simulink model "test_motion_controller"  (R2025a)
settings: Solver=FixedStepAuto  StartTime=0.0  StopTime=5  RelTol=1e-3
model workspace (MAT data in the model file):
  InitConfParams = Simulink.Parameter
  InitConfParams.Value.thresholds.jntVelMax = 40000
  InitConfParams.Value.thresholds.motorNominalCurrents = 0.34999999404
  InitConfParams.Value.thresholds.motorPeakCurrents = 0.699999988079
  InitConfParams.Value.thresholds.motorOverloadCurrents = 1
  InitConfParams.Value.thresholds.motorPwmLimit = 32000
  InitConfParams.Value.thresholds.motorCriticalTemperature = 0
  InitConfParams.Value.pids.currentPID.type : enumeration (value not decoded)
  InitConfParams.Value.pids.currentPID.OutMax = 0
  InitConfParams.Value.pids.currentPID.OutMin = 0
  InitConfParams.Value.pids.currentPID.P = 2
  InitConfParams.Value.pids.currentPID.I = 500
  InitConfParams.Value.pids.currentPID.D = 0
  InitConfParams.Value.pids.currentPID.N = 10
  InitConfParams.Value.pids.currentPID.I0 = 0
  InitConfParams.Value.pids.currentPID.D0 = 0
  InitConfParams.Value.pids.currentPID.shift_factor = 0
  InitConfParams.Value.pids.velocityPID.type : enumeration (value not decoded)
  InitConfParams.Value.pids.velocityPID.OutMax = 0
  InitConfParams.Value.pids.velocityPID.OutMin = 0
  InitConfParams.Value.pids.velocityPID.P = -20
  InitConfParams.Value.pids.velocityPID.I = -20
  InitConfParams.Value.pids.velocityPID.D = 0
  InitConfParams.Value.pids.velocityPID.N = 100
  InitConfParams.Value.pids.velocityPID.I0 = 0
  InitConfParams.Value.pids.velocityPID.D0 = 0
  InitConfParams.Value.pids.velocityPID.shift_factor = 10
  InitConfParams.Value.pids.positionPID.type : enumeration (value not decoded)
  InitConfParams.Value.pids.positionPID.OutMax = 0
  InitConfParams.Value.pids.positionPID.OutMin = 0
  InitConfParams.Value.pids.positionPID.P = 0
  InitConfParams.Value.pids.positionPID.I = 0
  InitConfParams.Value.pids.positionPID.D = 0
  InitConfParams.Value.pids.positionPID.N = 0
  InitConfParams.Value.pids.positionPID.I0 = 0
  InitConfParams.Value.pids.positionPID.D0 = 0
  InitConfParams.Value.pids.positionPID.shift_factor = 0
  InitConfParams.Value.motor.externals.enable_verbosity = 0
  InitConfParams.Value.motor.externals.has_hall_sens = 1
  InitConfParams.Value.motor.externals.has_quadrature_encoder = 0
  InitConfParams.Value.motor.externals.has_speed_quadrature_encoder = 0
  InitConfParams.Value.motor.externals.has_temperature_sens = 0
  InitConfParams.Value.motor.externals.encoder_tolerance = 0
  InitConfParams.Value.motor.externals.pole_pairs = 7
  InitConfParams.Value.motor.externals.rotor_encoder_resolution = 0
  InitConfParams.Value.motor.externals.rotor_index_offset = 0
  InitConfParams.Value.motor.externals.use_index = 0
  InitConfParams.Value.motor.Kbemf = 0
  InitConfParams.Value.motor.Rphase = 0
  InitConfParams.Value.motor.Imin = 0
  InitConfParams.Value.motor.Imax = 0
  InitConfParams.Value.motor.Vmax = 24
  InitConfParams.Value.motor.resistance = 25.8999996185
  InitConfParams.Value.motor.inductance = 271
  InitConfParams.Value.motor.thermal_resistance = 16
  InitConfParams.Value.motor.thermal_time_constant = 797.5
  InitConfParams.Value.motor.hall_sensors_offset = 30
  InitConfParams.Complexity = 'real'
  InitConfParams.Dimensions = [1 1]
  InitConfParams.DataType = 'Bus: ActuatorConfiguration'
undefined symbols (not defined in the file): ControlModes, EventTypes
settings Model: DataDictionary=embeddedBoard_common.sldd  Creator=mfussi  LastModifiedBy=mfussi
settings SolverCC: ConcurrentTasks=on  AutoInsertRateTranBlk=on
settings DataIOCC: SaveOutput=off  DSMLogging=off  SaveTime=off
settings OptimizationCC: DefaultParameterBehavior=Inlined  EnhancedBackFolding=on  PassReuseOutputArgsAs=Individual arguments  ZeroExternalMemoryAtStartup=off  ZeroInternalMemoryAtStartup=off  SimCompilerOptimization=on  OptimizeBlockOrder=speed  DifferentSizesBufferReuse=on  OptimizationCustomize=off  EfficientTunableParamExpr=on
settings DebuggingCC: ParameterPrecisionLossMsg=none  ParameterTunabilityLossMsg=error
settings ModelReferenceCC: SupportModelReferenceSimTargetCustomCode=on
settings SFSimCC: MATLABDynamicMemAlloc=off  SimTargetLang=C++  SimDLTargetLibrary=mkl-dnn
settings RTWCC: SystemTargetFile=ert.tlc  TemplateMakefile=ert_default_tmf  GPUComputeCapability=3.5  Description=Embedded Coder
settings CodeAppCC: ForceParamTrailComments=on  IgnoreCustomStorageClasses=off  MaxIdLength=95.0  OperatorAnnotations=on  SimulinkDataObjDesc=on  SFDataObjDesc=on  InsertBlockDesc=on
settings ERTTargetCC: ExtModeTransport=0.0  ExtModeStaticAlloc=off  ExtModeMexFile=ext_comm  ExtModeIntrfLevel=Level1  ERTCustomFileTemplate=example_file_process.tlc  TargetLangStandard=C99 (ISO)  GenerateSampleERTMain=on

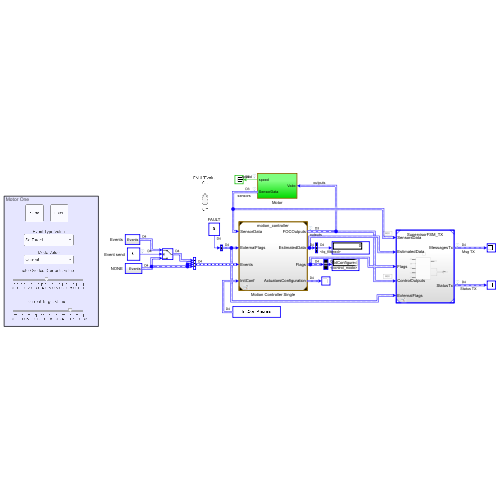
[thumbnail: Simulink's stored preview of the top-level diagram]
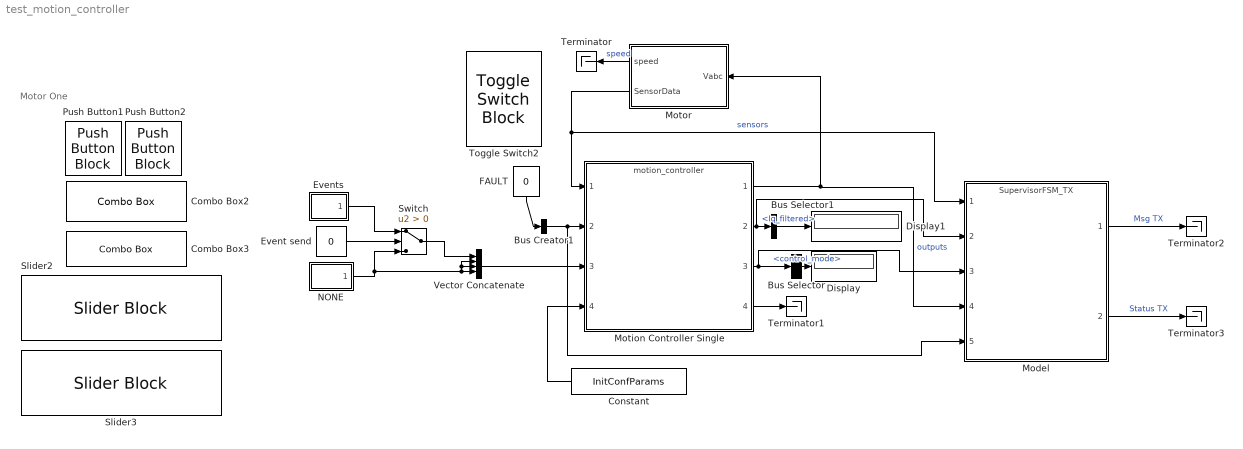
== system test_motion_controller ==
  note: Motor One
  Bus Creator1 : BusCreator  Inputs=1  OutDataTypeStr=Bus: ExternalFlags  NonVirtualBus=on
      settings: InheritFromInputs=off
  Bus Selector : BusSelector  OutputSignals=control_mode
  Bus Selector1 : BusSelector  OutputSignals=Iq_filtered
  Combo Box2 : ComboBox  SelectedLabel=SetTarget  UseEnumeratedDataType=on  EnumeratedDataType=EventTypes
  Combo Box3 : ComboBox  SelectedLabel=Current  UseEnumeratedDataType=on  EnumeratedDataType=ControlModes
  Constant : Constant  Value=InitConfParams  OutDataTypeStr=Bus: ActuatorConfiguration  SampleTime=1e-3
  Display : Display
  Display1 : Display
  Event send : Constant  Value=0  OutDataTypeStr=boolean  SampleTime=1e-3
  Events : Subsystem
  FAULT : Constant  Value=0  OutDataTypeStr=Inherit: Inherit via back propagation  SampleTime=0.001
  Model : ModelReference  ModelNameDialog=SupervisorFSM_TX.slx  SimulationMode=Normal  ModelReferenceVersion=10.14
  Motion Controller Single : ModelReference  ModelNameDialog=motion_controller.slx  ModelReferenceVersion=5.2
  Motor : Subsystem
  NONE : Subsystem
  Push Button1 : PushButtonBlock  ButtonText=Send  IconOnColor=[0.0, 0.39215686274509803, 0.0]  IconOffColor=[0.0, 1.0, 0.0]  OffValue=0.000000
  Push Button2 : PushButtonBlock  ButtonText=Latch  ButtonType=Latch  IconOnColor=[0.0, 0.39215686274509803, 0.0]  IconOffColor=[0.0, 1.0, 0.0]  OffValue=0.000000
  Slider2 : SliderBlock  ScaleMax=1
  Slider3 : SliderBlock  ScaleMax=0.36
  Switch : Switch  Criteria=u2 > Threshold  SaturateOnIntegerOverflow=off  InputSameDT=off
  Terminator{,1..3} (4 alike) : Terminator
  Toggle Switch2 : ToggleSwitchBlock
  Vector Concatenate : Concatenate  NumInputs=4
  wires:
  Bus Selector/1 -> Display/1  "<control_mode>"
  Motion Controller Single/2 -> Model/2, Bus Selector1/1
  Bus Creator1/1 -> Model/5, Motion Controller Single/2
  Motor/2(SensorData) -> Motion Controller Single/1, Model/1  "sensors"
  Motion Controller Single/1 -> Motor/1(Vabc), Model/4  "outputs"
  Switch/1 -> Vector Concatenate/1
  FAULT/1 -> Bus Creator1/1
  Bus Selector1/1 -> Display1/1  "<Iq_filtered>"
  NONE/1(Events) -> Vector Concatenate/3, Vector Concatenate/2, Vector Concatenate/4, Switch/3
  Events/1(Events) -> Switch/1
  Motor/1(speed) -> Terminator/1  "speed"
  Constant/1 -> Motion Controller Single/4
  Motion Controller Single/3 -> Model/3, Bus Selector/1
  Motion Controller Single/4 -> Terminator1/1
  Model/1 -> Terminator2/1  "Msg TX"
  Model/2 -> Terminator3/1  "Status TX"
  Vector Concatenate/1 -> Motion Controller Single/3
  Event send/1 -> Switch/2

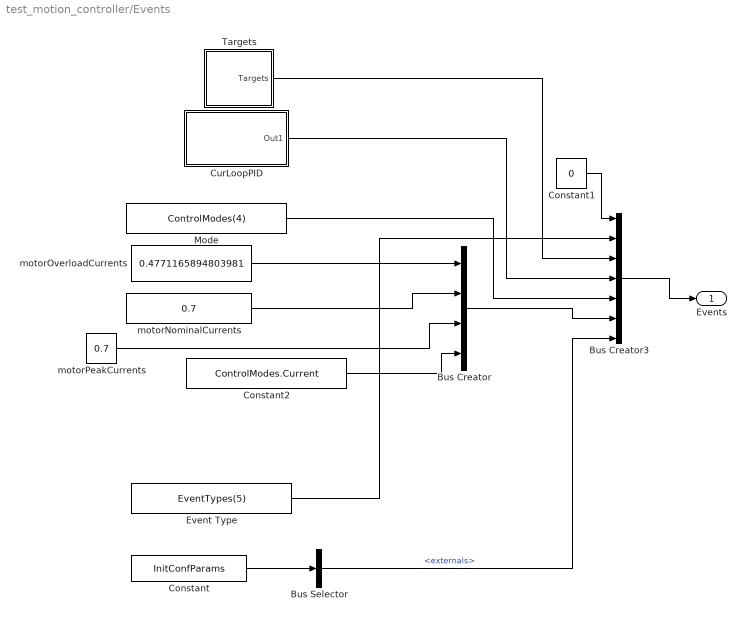
== system test_motion_controller/Events ==
  Bus Creator : BusCreator  Inputs=4  OutDataTypeStr=Bus: SupervisorInputLimits  NonVirtualBus=on
      settings: InheritFromInputs=off
  Bus Creator3 : BusCreator  Inputs=7  OutDataTypeStr=Bus: ReceivedEvents  NonVirtualBus=on
      settings: InheritFromInputs=off
  Bus Selector : BusSelector  OutputSignals=motor.externals
  Constant : Constant  Value=InitConfParams  OutDataTypeStr=Bus: ActuatorConfiguration
  Constant1 : Constant  Value=0  OutDataTypeStr=uint8
  Constant2 : Constant  Value=ControlModes.Current  OutDataTypeStr=Enum: ControlModes
  CurLoopPID : Subsystem  mask{OutMax=0, OutMin=0, P=20, I=5000, D=0, N=10, I0=0, D0=0, shift_factor=0}
      mask prompts: shift_factor "Shift Factor"
  Event Type : Constant  Value=EventTypes(5)  OutDataTypeStr=Enum: EventTypes
  Mode : Constant  Value=ControlModes(4)  OutDataTypeStr=Enum: ControlModes
  Targets : Subsystem
  motorNominalCurrents : Constant  Value=0.7  OutDataTypeStr=single
  motorOverloadCurrents : Constant  Value=0.4771165894803981  OutDataTypeStr=single
  motorPeakCurrents : Constant  Value=0.7  OutDataTypeStr=single
  Events : Outport  OutDataTypeStr=Bus: ReceivedEvents
  wires:
  motorPeakCurrents/1 -> Bus Creator/3
  Constant2/1 -> Bus Creator/4
  motorOverloadCurrents/1 -> Bus Creator/1
  motorNominalCurrents/1 -> Bus Creator/2
  Bus Creator3/1 -> Events/1
  Constant/1 -> Bus Selector/1
  Bus Selector/1 -> Bus Creator3/7  "<externals>"
  Bus Creator/1 -> Bus Creator3/6
  Mode/1 -> Bus Creator3/5
  CurLoopPID/1(Out1) -> Bus Creator3/4
  Targets/1(Targets) -> Bus Creator3/3
  Event Type/1 -> Bus Creator3/2
  Constant1/1 -> Bus Creator3/1

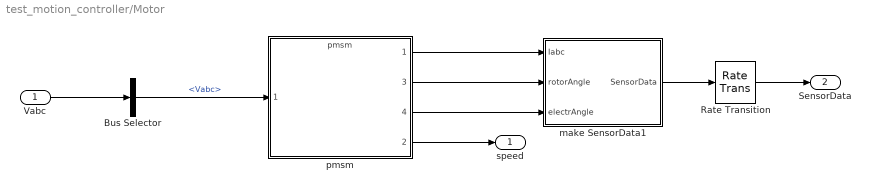
== system test_motion_controller/Motor ==
  Vabc : Inport
  Bus Selector : BusSelector  OutputSignals=Vabc
  Rate Transition : RateTransition  Integrity=off  OutPortSampleTime=Ts_ControlFOC
  make SensorData1 : Subsystem
  pmsm : ModelReference  ModelNameDialog=pmsm.slx  SimulationMode=Normal  ModelReferenceVersion=10.2
      settings: PortSchema="{\"entries\":[{\"content\":{\"sides\":[{\"content\":{\"connectorIds\":[\"In1\"]},\"type\":\"ConnectorPlacement.EquallySpacedRectSide\",\"uuid\":\"8cec65a8-4219-41d1-959d-4e8d996cc561\"},{\"content\":{\"connectorIds\":[\"Out1\",\"Out3\",\"Out4\",\"Out2\"],\"side\":\"RIGHT\"},\"type\":\"ConnectorPlacement.EquallySpacedRectSide\",\"uuid\":\"120dfdfb-4ec8-4266-9e58-5a4f10fe78d1\"},{\"content\":{\"side\":\"TOP\"},\"type\":\"ConnectorPlacement.EquallySpacedRectSide\",\"uuid\":\"6d35c191-eb3f-4663-84d3-c95352a14c82\"}]},\"type\":\"ConnectorPlacement.EquallySpacedConnector\",\"uuid\":\"bf10708e-bbfb-4369-9195-0995d9345086\"}],\"packageUris\":[\"http://schema.mathworks.com/mf0/Connector/R2020b\"],\"version\":\"1.0\"}"
  speed : Outport
  SensorData : Outport  Port=2
  wires:
  make SensorData1/1(SensorData) -> Rate Transition/1
  pmsm/1 -> make SensorData1/1(Iabc)
  Bus Selector/1 -> pmsm/1  "<Vabc>"
  Vabc/1 -> Bus Selector/1
  Rate Transition/1 -> SensorData/1
  pmsm/4 -> make SensorData1/3(electrAngle)
  pmsm/2 -> speed/1
  pmsm/3 -> make SensorData1/2(rotorAngle)

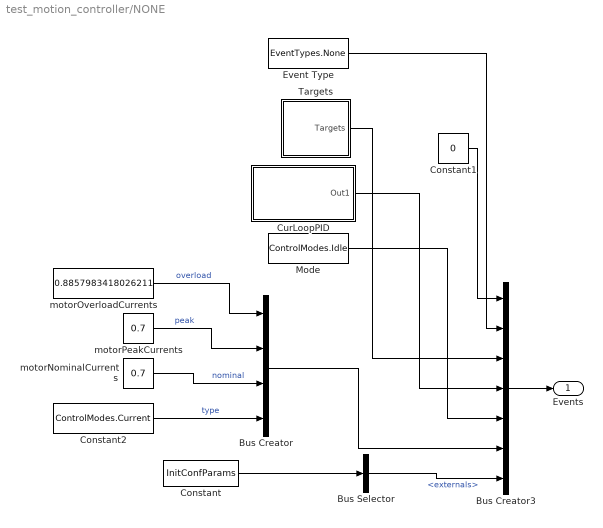
== system test_motion_controller/NONE ==
  Bus Creator : BusCreator  Inputs=4  OutDataTypeStr=Bus: SupervisorInputLimits
  Bus Creator3 : BusCreator  Inputs=7  OutDataTypeStr=Bus: ReceivedEvents  NonVirtualBus=on
      settings: InheritFromInputs=off
  Bus Selector : BusSelector  OutputSignals=motor.externals
  Constant : Constant  Value=InitConfParams  OutDataTypeStr=Bus: ActuatorConfiguration
  Constant1 : Constant  Value=0  OutDataTypeStr=uint8
  Constant2 : Constant  Value=ControlModes.Current  OutDataTypeStr=Enum: ControlModes
  CurLoopPID : Subsystem  mask{OutMax=0, OutMin=0, P=2, I=500, D=0, N=10, I0=0, D0=0, shift_factor=0}
      mask prompts: shift_factor "Shift Factor"
  Event Type : Constant  Value=EventTypes.None  OutDataTypeStr=Enum: EventTypes
  Mode : Constant  Value=ControlModes.Idle  OutDataTypeStr=Enum: ControlModes
  Targets : Subsystem
  motorNominalCurrents : Constant  Value=0.7  OutDataTypeStr=single
  motorOverloadCurrents : Constant  Value=0.8857983418026211  OutDataTypeStr=single
  motorPeakCurrents : Constant  Value=0.7  OutDataTypeStr=single
  Events : Outport  OutDataTypeStr=Bus: ReceivedEvents
  wires:
  motorNominalCurrents/1 -> Bus Creator/3  "nominal"
  motorOverloadCurrents/1 -> Bus Creator/1  "overload"
  motorPeakCurrents/1 -> Bus Creator/2  "peak"
  Bus Creator3/1 -> Events/1
  Constant/1 -> Bus Selector/1
  Constant2/1 -> Bus Creator/4  "type"
  Bus Selector/1 -> Bus Creator3/7  "<externals>"
  Bus Creator/1 -> Bus Creator3/6
  Mode/1 -> Bus Creator3/5
  CurLoopPID/1(Out1) -> Bus Creator3/4
  Targets/1(Targets) -> Bus Creator3/3
  Event Type/1 -> Bus Creator3/2
  Constant1/1 -> Bus Creator3/1

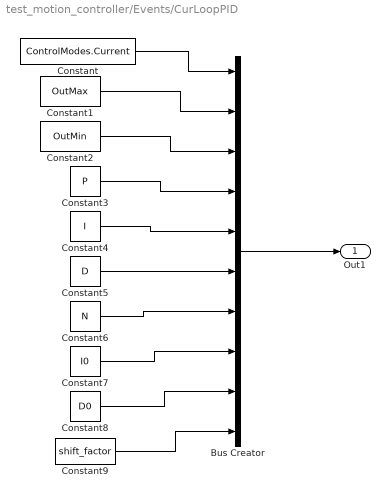
== system test_motion_controller/Events/CurLoopPID ==
  Bus Creator : BusCreator  Inputs=10  OutDataTypeStr=Bus: PID  NonVirtualBus=on
      settings: InheritFromInputs=off
  Constant : Constant  Value=ControlModes.Current
  Constant1 : Constant  Value=OutMax  OutDataTypeStr=single
  Constant2 : Constant  Value=OutMin  OutDataTypeStr=single
  Constant3 : Constant  Value=P  OutDataTypeStr=single
  Constant4 : Constant  Value=I  OutDataTypeStr=single
  Constant5 : Constant  Value=D  OutDataTypeStr=single
  Constant6 : Constant  Value=N  OutDataTypeStr=single
  Constant7 : Constant  Value=I0  OutDataTypeStr=single
  Constant8 : Constant  Value=D0  OutDataTypeStr=single
  Constant9 : Constant  Value=shift_factor  OutDataTypeStr=uint8
  Out1 : Outport  OutDataTypeStr=Bus: PID
  wires:
  Bus Creator/1 -> Out1/1
  Constant8/1 -> Bus Creator/9
  Constant3/1 -> Bus Creator/4
  Constant5/1 -> Bus Creator/6
  Constant1/1 -> Bus Creator/2
  Constant7/1 -> Bus Creator/8
  Constant2/1 -> Bus Creator/3
  Constant9/1 -> Bus Creator/10
  Constant4/1 -> Bus Creator/5
  Constant/1 -> Bus Creator/1
  Constant6/1 -> Bus Creator/7

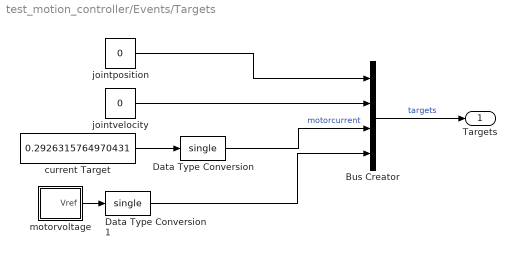
== system test_motion_controller/Events/Targets ==
  Bus Creator : BusCreator  Inputs=4  OutDataTypeStr=Bus: Targets  NonVirtualBus=on
      settings: InheritFromInputs=off
  Data Type Conversion : DataTypeConversion  OutDataTypeStr=single  SaturateOnIntegerOverflow=off  RndMeth=Floor
  Data Type Conversion1 : DataTypeConversion  OutDataTypeStr=single  SaturateOnIntegerOverflow=off  RndMeth=Floor
  current Target : Constant  Value=0.2926315764970431
  jointposition : Constant  Value=0  OutDataTypeStr=single
  jointvelocity : Constant  Value=0  OutDataTypeStr=single
  motorvoltage : Subsystem
  Targets : Outport
  wires:
  Bus Creator/1 -> Targets/1  "targets"
  jointposition/1 -> Bus Creator/1
  jointvelocity/1 -> Bus Creator/2
  Data Type Conversion1/1 -> Bus Creator/4
  Data Type Conversion/1 -> Bus Creator/3  "motorcurrent"
  motorvoltage/1(Vref) -> Data Type Conversion1/1
  current Target/1 -> Data Type Conversion/1

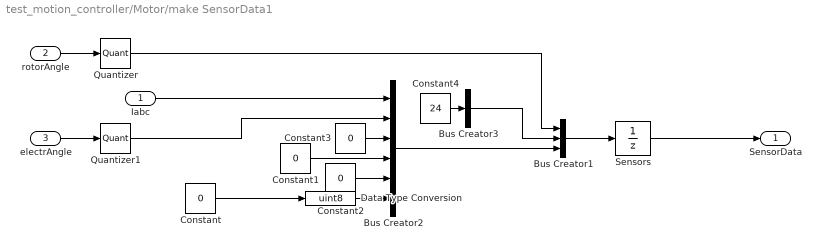
== system test_motion_controller/Motor/make SensorData1 ==
  Iabc : Inport
  rotorAngle : Inport  Port=2
  electrAngle : Inport  Port=3
  Bus Creator1 : BusCreator  Inputs=3  OutDataTypeStr=Bus: SensorsData  NonVirtualBus=on
      settings: InheritFromInputs=off
  Bus Creator2 : BusCreator  Inputs=6  OutDataTypeStr=Bus: MotorSensors  NonVirtualBus=on
      settings: InheritFromInputs=off
  Bus Creator3 : BusCreator  Inputs=1  OutDataTypeStr=Bus: DriverSensors  NonVirtualBus=on
      settings: InheritFromInputs=off
  Constant{,1..3} (4 alike) : Constant  Value=0  OutDataTypeStr=single
  Constant4 : Constant  Value=24  OutDataTypeStr=single
  Data Type Conversion : DataTypeConversion  OutDataTypeStr=uint8  SaturateOnIntegerOverflow=off  RndMeth=Floor
  Quantizer : Quantizer  QuantizationInterval=60
  Quantizer1 : Quantizer  QuantizationInterval=60
  Sensors : UnitDelay  SampleTime=-1  HasFrameUpgradeWarning=on
  SensorData : Outport
  wires:
  Sensors/1 -> SensorData/1
  Constant/1 -> Data Type Conversion/1
  Iabc/1 -> Bus Creator2/1
  rotorAngle/1 -> Quantizer/1
  Bus Creator1/1 -> Sensors/1
  electrAngle/1 -> Quantizer1/1
  Data Type Conversion/1 -> Bus Creator2/6
  Constant1/1 -> Bus Creator2/4
  Constant2/1 -> Bus Creator2/5
  Constant3/1 -> Bus Creator2/3
  Bus Creator3/1 -> Bus Creator1/2
  Bus Creator2/1 -> Bus Creator1/3
  Constant4/1 -> Bus Creator3/1
  Quantizer/1 -> Bus Creator1/1
  Quantizer1/1 -> Bus Creator2/2

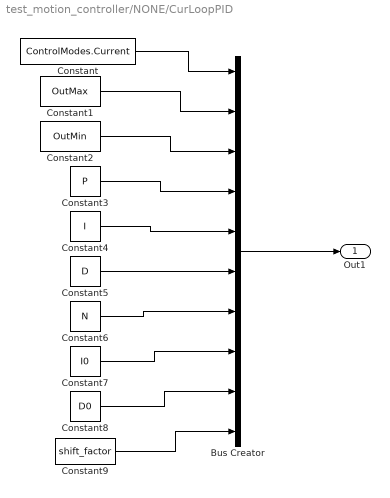
== system test_motion_controller/NONE/CurLoopPID ==
  Bus Creator : BusCreator  Inputs=10  OutDataTypeStr=Bus: PID  NonVirtualBus=on
      settings: InheritFromInputs=off
  Constant : Constant  Value=ControlModes.Current
  Constant1 : Constant  Value=OutMax  OutDataTypeStr=single
  Constant2 : Constant  Value=OutMin  OutDataTypeStr=single
  Constant3 : Constant  Value=P  OutDataTypeStr=single
  Constant4 : Constant  Value=I  OutDataTypeStr=single
  Constant5 : Constant  Value=D  OutDataTypeStr=single
  Constant6 : Constant  Value=N  OutDataTypeStr=single
  Constant7 : Constant  Value=I0  OutDataTypeStr=single
  Constant8 : Constant  Value=D0  OutDataTypeStr=single
  Constant9 : Constant  Value=shift_factor  OutDataTypeStr=uint8
  Out1 : Outport  OutDataTypeStr=Bus: PID
  wires:
  Bus Creator/1 -> Out1/1
  Constant8/1 -> Bus Creator/9
  Constant3/1 -> Bus Creator/4
  Constant5/1 -> Bus Creator/6
  Constant1/1 -> Bus Creator/2
  Constant7/1 -> Bus Creator/8
  Constant2/1 -> Bus Creator/3
  Constant9/1 -> Bus Creator/10
  Constant4/1 -> Bus Creator/5
  Constant/1 -> Bus Creator/1
  Constant6/1 -> Bus Creator/7

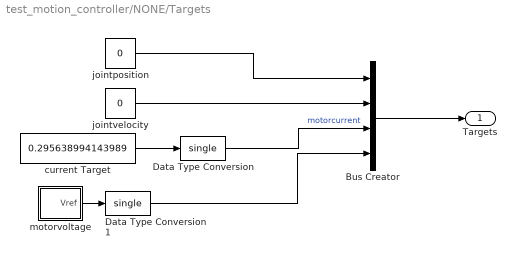
== system test_motion_controller/NONE/Targets ==
  Bus Creator : BusCreator  Inputs=4  OutDataTypeStr=Bus: Targets  NonVirtualBus=on
      settings: InheritFromInputs=off
  Data Type Conversion : DataTypeConversion  OutDataTypeStr=single  SaturateOnIntegerOverflow=off  RndMeth=Floor
  Data Type Conversion1 : DataTypeConversion  OutDataTypeStr=single  SaturateOnIntegerOverflow=off  RndMeth=Floor
  current Target : Constant  Value=0.295638994143989
  jointposition : Constant  Value=0  OutDataTypeStr=single
  jointvelocity : Constant  Value=0  OutDataTypeStr=single
  motorvoltage : Subsystem
  Targets : Outport
  wires:
  Bus Creator/1 -> Targets/1
  jointposition/1 -> Bus Creator/1
  jointvelocity/1 -> Bus Creator/2
  Data Type Conversion1/1 -> Bus Creator/4
  Data Type Conversion/1 -> Bus Creator/3  "motorcurrent"
  motorvoltage/1(Vref) -> Data Type Conversion1/1
  current Target/1 -> Data Type Conversion/1

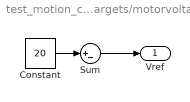
== system test_motion_controller/Events/Targets/motorvoltage ==
  Constant : Constant  Value=20
  Sum : Sum  Inputs=|+-
  Vref : Outport
  wires:
  Sum/1 -> Vref/1
  Constant/1 -> Sum/1

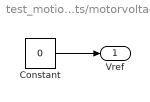
== system test_motion_controller/NONE/Targets/motorvoltage ==
  Constant : Constant  Value=0
  Vref : Outport
  wires:
  Constant/1 -> Vref/1
